simulink model "lab2simulink_1"  (R2024b)
settings: Solver=VariableStepAuto  StartTime=0.0  StopTime=10.0  RelTol=1e-3
settings Model: Creator=ttkim2  LastModifiedBy=ttkim2

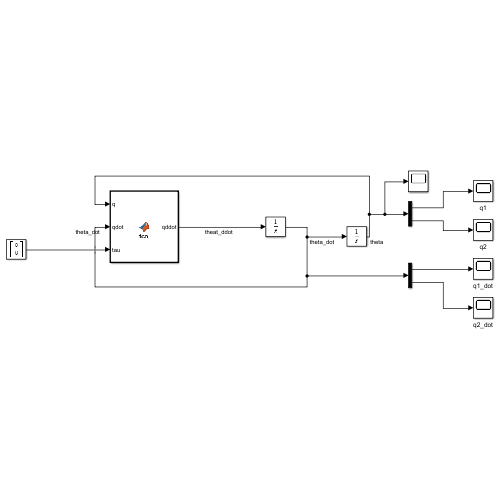
[thumbnail: Simulink's stored preview of the top-level diagram]
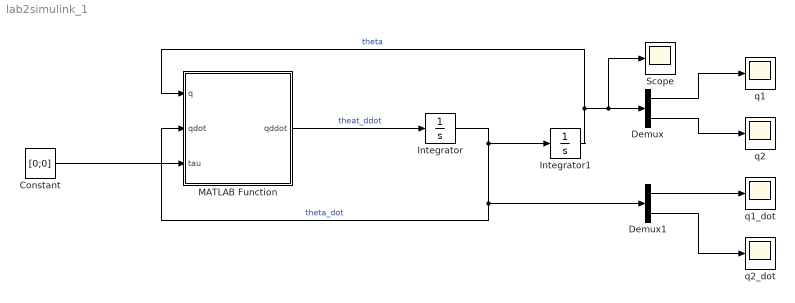
== system lab2simulink_1 ==
  Constant : Constant  Value=[0;0]  VectorParams1D=off
  Demux : Demux  Outputs=2
  Demux1 : Demux  Outputs=2
  Integrator : Integrator  InitialCondition=[0;0]
  Integrator1 : Integrator  InitialCondition=[pi/2; 0]
  MATLAB Function : MATLAB Function  TreatAsAtomicUnit=on
  Scope : Scope
  q1 : Scope
  q1_dot : Scope
  q2 : Scope
  q2_dot : Scope
  wires:
  Integrator1/1 -> Scope/1, Demux/1, MATLAB Function/1(q)  "theta"
  Integrator/1 -> Demux1/1, MATLAB Function/2(qdot), Integrator1/1  "theta_dot"
  Demux1/1 -> q1_dot/1
  Demux/2 -> q2/1
  Demux/1 -> q1/1
  MATLAB Function/1(qddot) -> Integrator/1  "theat_ddot"
  Demux1/2 -> q2_dot/1
  Constant/1 -> MATLAB Function/3(tau)

== matlab function lab2simulink_1/MATLAB Function ==
  data: q input; qddot output; qdot input; tau input
function qddot = fcn(q, qdot, tau)
p1 = 0.03;
p2 = 0.0128;
p3 = 0.0076;
p4 = 0.0753;
p5 = 0.0298;
g  = 9.81;


theta2  = q(1);
dtheta2 = qdot(1);
theta3  = q(2);
dtheta3 = qdot(2);

d = theta3 - theta2;

D = [ p1,           -p3*sin(d);
     -p3*sin(d),     p2      ];

C = [ 0,                 -p3*cos(d)*dtheta3;
      p3*cos(d)*dtheta2,  0               ];

G = [ -p4*g*sin(theta2);
      -p5*g*cos(theta3) ];


qddot = (inv(D)*tau - inv(D)*C*qdot - inv(D)*G);
